simulink library "Yaw_Motor_Lib"  (R2025a)
settings: Solver=ode45  StartTime=0.0  StopTime=10.0  RelTol=1e-3  EnableMultiTasking=on
undefined symbols (not defined in the file): WT_Params
libraries: fl_lib x6, nesl_utility x5, ee_lib x1, sdl_lib x1, Yaw_Gearbox_Lib x1
Description:
  | Copyright 2009-2025 The MathWorks, Inc. MathWorks, Inc.
settings Model: Creator=smiller  LastModifiedBy=smiller
settings SolverCC: AlgebraicLoopSolver=TrustRegion
settings DataIOCC: LimitDataPoints=on  SaveFormat=Array  SignalLoggingSaveFormat=ModelDataLogs  ReturnWorkspaceOutputs=off
settings OptimizationCC: ReuseModelBlockBuffer=off  ExpressionDepthLimit=2147483647.0  LifeSpan=inf
settings DebuggingCC: UnderspecifiedInitializationDetection=Classic  MergeDetectMultiDrivingBlocksExec=none  SolverPrmCheckMsg=warning  FcnCallInpInsideContextMsg=warning  UnconnectedInputMsg=warning  UnconnectedOutputMsg=warning  UnconnectedLineMsg=warning  AllowSymbolicDim=off  StateNameClashWarn=warning  PregeneratedLibrarySubsystemCodeDiagnostic=none  SFUnexpectedBacktrackingDiag=warning  SFNoUnconditionalDefaultTransitionDiag=warning  SFExecutionAtInitializationDiag=none  ArithmeticOperatorsInVariantConditions=warning
settings HardwareCC: ProdBitPerPointer=32.0  ProdBitPerSizeT=32.0  ProdBitPerPtrDiffT=32.0  ProdLargestAtomicFloat=None  ProdIntDivRoundTo=Undefined  ProdEndianess=Unspecified  ProdWordSize=32.0  ProdHWDeviceType=32-bit Generic
settings ModelReferenceCC: EnableRefExpFcnMdlSchedulingChecks=on  PropagateSignalLabelsOutOfModel=off
settings SFSimCC: SimUseLocalCustomCode=off  CustomCodeUndefinedFunction=UseInterfaceOnly
settings RTWCC: RTWUseLocalCustomCode=off  GPUComputeCapability=3.5  DLArmComputeVersion=19.05
settings CodeAppCC: StateflowObjectComments=on
settings GRTTargetCC: TargetLangStandard=C89/C90 (ANSI)  CombineOutputUpdateFcns=off  GRTInterface=on
settings ConfigComp: CovMetricSettings=dw  CovSaveCumulativeToWorkspaceVar=on  CovSaveSingleToWorkspaceVar=on  CovExternalEMLEnable=off  CovSFcnEnable=off

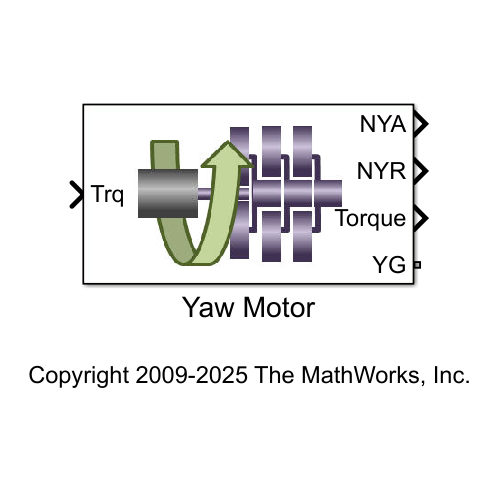
[thumbnail: Simulink's stored preview of the top-level diagram]
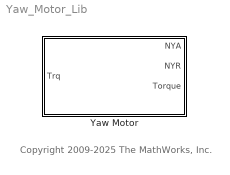
== system Yaw_Motor_Lib ==
  note: Copyright 2009-2025 The MathWorks, Inc.
  Yaw Motor : Subsystem
      mask Display: image('Yaw_Servomotor_Horizontal_IMAGE.jpg');

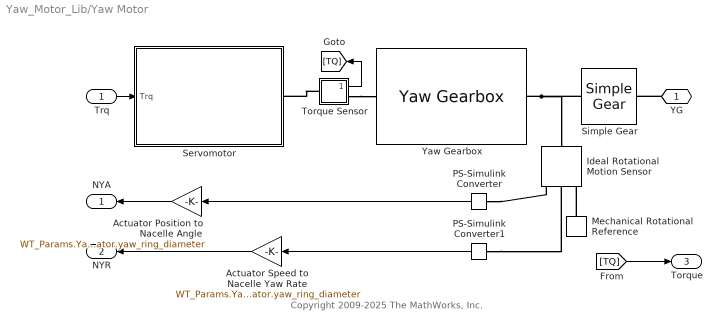
== system Yaw_Motor_Lib/Yaw Motor ==
  note: Copyright 2009-2025 The MathWorks, Inc.
  Trq : Inport
  Actuator Position to Nacelle Angle : Gain  Gain=WT_Params.Yaw_Actuator.yaw_gear_diameter/WT_Params.Yaw_Actuator.yaw_ring_diameter
  Actuator Speed to Nacelle Yaw Rate : Gain  Gain=WT_Params.Yaw_Actuator.yaw_gear_diameter/WT_Params.Yaw_Actuator.yaw_ring_diameter
  Ideal Rotational Motion Sensor : fl_lib/Mechanical/Mechanical Sensors/Ideal Rotational Motion Sensor  reference=foundation.enum.MeasurementReference.difference  acceleration_port=false  velocity_port=true  position_port=true  wrap_angle=simscape.enum.onoff.off  offset=0 rad
  Mechanical Rotational Reference : fl_lib/Mechanical/Rotational Elements/Mechanical Rotational Reference
  PS-Simulink Converter : nesl_utility/PS-Simulink Converter  PhysicalDomain=network_engine_domain  SubClassName=ps_output  LeftPortType=input  RightPortType=output  PseudoPeriodic=off  Frequencies=[]  VectorFormat=1-D array  Unit=deg  AffineConversion=off
  PS-Simulink Converter1 : nesl_utility/PS-Simulink Converter  PhysicalDomain=network_engine_domain  SubClassName=ps_output  LeftPortType=input  RightPortType=output  PseudoPeriodic=off  Frequencies=[]  VectorFormat=1-D array  Unit=deg/s  AffineConversion=off
  Servomotor : Subsystem
      mask Display: image(imread('Yaw_Servomotor_IMAGE.jpg'));
  Simple Gear : sdl_lib/Gears/Simple Gear  ratio=1/(WT_Params.Yaw_Actuator.yaw_gear_diameter/WT_Params.Yaw_Actuator.yaw_ring_diameter)  rotation_direction=3-2*(2)  friction_model=1  T_noload=0.1 N*m  T_nom=5 N*m  efficiency_nom=0.8  efficiency=0.8  temperature_TLU=[ 280 300 320 ] K  load_TLU=[ 1 5 10 ] N*m  efficiency_TLU=[ 0.95 0.9 0.85 ]  efficiency_TLU2=[ 0.85 0.8 0.75; 0.95 0.9 0.85; 0.85 0.8 0.7 ]  w_thr=0.01 rad/s  pwr_thr=0.001 W  enable_backlash=false  hardstop_model=simscape.enum.hardstop.smooth  backlash_distance=1e-3 mm  r_base=0.1 m  transition=1e-4 mm  backlash_stiffness=1e7 N/m  backlash_damping=1e6 N*s/m  coeff_rest=0  v_tol=0.001 m/s  f_tol=0 N  mu_visc=[ 0 0 ] N*m/(rad/s)  thermal_mass=50 J/K  temperature_specify=off  temperature_priority=High  temperature=300 K  temperature_nominal_specify=off  temperature_nominal_value=1  temperature_nominal_unit=K  x_backlash_specify=off  x_backlash_priority=None  x_backlash=0 mm  x_backlash_nominal_specify=off  x_backlash_nominal_value=1  x_backlash_nominal_unit=mm  f_hardstop_specify=off  f_hardstop_priority=None  f_hardstop=0 N  f_hardstop_nominal_specify=off  f_hardstop_nominal_value=1  f_hardstop_nominal_unit=N  v_backlash_specify=off  v_backlash_priority=None  v_backlash=0 m/s  v_backlash_nominal_specify=off  v_backlash_nominal_value=1  v_backlash_nominal_unit=m/s
  Torque Sensor : Subsystem
      mask Display: disp('S')
  Yaw Gearbox : Yaw_Gearbox_Lib/Yaw Gearbox  SystemSampleTime=-1  VariantActivationTime=update diagram  EmptyChoice=off  PassThrough=off  PassThroughVariantControl=(default)  EmptyChoiceVariantControl=(default)  AllowFlexibleInterface=on  Latency=0  AutoFrameSizeCalculation=off
  YG : PMIOPort  Side=Right
  NYA : Outport  VectorParamsAs1DForOutWhenUnconnected=off
  NYR : Outport  Port=2  VectorParamsAs1DForOutWhenUnconnected=off
  Torque : Outport  Port=3  VectorParamsAs1DForOutWhenUnconnected=off
  wires:
  PS-Simulink Converter1/1 -> Actuator Speed to Nacelle Yaw Rate/1
  PS-Simulink Converter/1 -> Actuator Position to Nacelle Angle/1
  [TQ] -> Torque/1
  Torque Sensor/1(Trq) -> [TQ]
  Actuator Speed to Nacelle Yaw Rate/1 -> NYR/1
  Actuator Position to Nacelle Angle/1 -> NYA/1
  Trq/1 -> Servomotor/1(Trq)
  connections:
  YG/RConn1 -- Simple Gear/RConn1
  PS-Simulink Converter/LConn1 -- Ideal Rotational Motion Sensor/RConn3
  Mechanical Rotational Reference/LConn1 -- Ideal Rotational Motion Sensor/RConn1
  PS-Simulink Converter1/LConn1 -- Ideal Rotational Motion Sensor/RConn2
  Yaw Gearbox/RConn1 -- Ideal Rotational Motion Sensor/LConn1 -- Simple Gear/LConn1
  Torque Sensor/RConn1 -- Yaw Gearbox/LConn1
  Torque Sensor/LConn1 -- Servomotor/RConn1

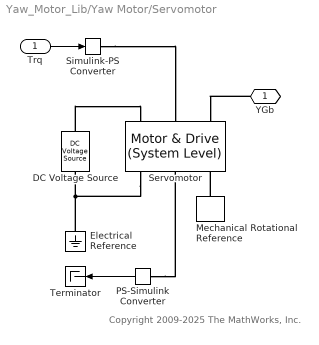
== system Yaw_Motor_Lib/Yaw Motor/Servomotor ==
  note: Copyright 2009-2025 The MathWorks, Inc.
  Trq : Inport
  DC Voltage Source : fl_lib/Electrical/Electrical Sources/DC Voltage Source  v0=WT_Params.Yaw_Actuator.Motor.voltage V
  Electrical Reference : fl_lib/Electrical/Electrical Elements/Electrical Reference
  Mechanical Rotational Reference : fl_lib/Mechanical/Rotational Elements/Mechanical Rotational Reference
  PS-Simulink Converter : nesl_utility/PS-Simulink Converter  PhysicalDomain=network_engine_domain  SubClassName=ps_output  LeftPortType=input  RightPortType=output  PseudoPeriodic=off  Frequencies=[]  VectorFormat=1-D array  Unit=deg/s  AffineConversion=off
  Servomotor : ee_lib/Electromechanical/Motor & Drive (System Level)  torque_speed_param=1  overtorque_param=ee.enum.electromech.overtorque.no  T_t=WT_Params.Yaw_Actuator.Motor.max_torque_vector N*m  T_t_intermittent=[.36, .32, .28, 0] N*m  T_t_2D=[.09, .09, .09; .08, .08, .08; .07, .07, .07; 0, 0, 0] N*m  T_t_intermittent_2D=[.36, .36, .36; .32, .32, .32; .28, .28, .28; 0, 0, 0] N*m  w_t=WT_Params.Yaw_Actuator.Motor.max_speed_vector rpm  vdc_t=[6, 12, 24] V  torque_max=0.1 N*m  power_max=30 W  torque_max_intermittent=0.4 N*m  power_max_intermittent=120 W  time_overtorque=30 s  time_recover=60 s  Tc=WT_Params.Yaw_Actuator.Motor.control_time_constant s  EnableSwitch=simscape.enum.onoff.off  losses_param=1  eff=100  w_eff=3.75e+03 rpm  T_eff=0.08 N*m  Piron=0 W  Pbase=0 W  w_eff_vec=[-8000 -4000 0 4000 8000] rpm  T_eff_vec=[0 0.03 0.06 0.09] N*m  v_eff_vec=[100, 250, 400] V  losses_mat=[1.49 1.67 2.21 3.10; 0.42 0.69 1.14 2.03; 0.06 0.24 0.78 1.68; 0.42 0.69 1.14 2.03; 1.49 1.67 2.21 3.10] W  efficiency_mat=[95 95 95 95; 95 95 95 95; 95 95 95 95; 95 95 95 95; 95 95 95 95]  losses_mat_3D=ones(5, 4, 3) W  efficiency_mat_3D=95 * ones(5, 4, 3)  Res=WT_Params.Yaw_Actuator.Motor.resistance Ohm  J=0 kg*m^2  lam=WT_Params.Yaw_Actuator.Motor.damping N*m/(rad/s)  speed0=0 rpm  faulted_specify=off  faulted_priority=None  faulted=0  faulted_nominal_specify=off  faulted_nominal_value=1  faulted_nominal_unit=1  isSwitchedOff_specify=off  isSwitchedOff_priority=None  isSwitchedOff=0  isSwitchedOff_nominal_specify=off  isSwitchedOff_nominal_value=1  isSwitchedOff_nominal_unit=1  torqueLimitContinuous_specify=off  torqueLimitContinuous_priority=None  torqueLimitContinuous=0 N*m  torqueLimitContinuous_nominal_specify=off  torqueLimitContinuous_nominal_value=1  torqueLimitContinuous_nominal_unit=N*m  alpha=3.93e-3 1/K  Tmeas=25 degC  Tmeas2=125 degC  losses_mat_T2=[1.49, 1.74, 2.49, 3.74; .42, .67, 1.42, 2.67; .06, .31, 1.06, 2.31; .42, .67, 1.42, 2.67; 1.49, 1.74, 2.49, 3.74] W  efficiency_mat_T2=[95, 95, 95, 95; 95, 95, 95, 95; 95, 95, 95, 95; 95, 95, 95, 95; 95, 95, 95, 95]  losses_mat_3D_T2=ones(5, 4, 3) W  efficiency_mat_3D_T2=95 * ones(5, 4, 3)  thermal_mass=100 J/K  initial_temperature=25 degC
  Simulink-PS Converter : nesl_utility/Simulink-PS Converter  PhysicalDomain=network_engine_domain  SubClassName=ps_input  LeftPortType=input  RightPortType=output  PseudoPeriodic=off  Frequencies=[]  NoiseDistribution=none  NoiseParameters=[]  Unit=1  AffineConversion=off  FilteringAndDerivatives=filter  SimscapeFilterOrder=1  InputFilterTimeConstant=0.005  UdotUserProvided=1
  Terminator : Terminator
  YGb : PMIOPort  Side=Right
  wires:
  Trq/1 -> Simulink-PS Converter/1
  PS-Simulink Converter/1 -> Terminator/1
  connections:
  YGb/RConn1 -- Servomotor/LConn3
  Simulink-PS Converter/RConn1 -- Servomotor/LConn2
  PS-Simulink Converter/LConn1 -- Servomotor/RConn2
  Mechanical Rotational Reference/LConn1 -- Servomotor/RConn3
  Electrical Reference/LConn1 -- DC Voltage Source/RConn1 -- Servomotor/RConn1
  DC Voltage Source/LConn1 -- Servomotor/LConn1

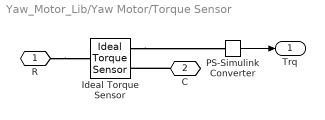
== system Yaw_Motor_Lib/Yaw Motor/Torque Sensor ==
  Ideal Torque Sensor : fl_lib/Mechanical/Mechanical Sensors/Ideal Torque Sensor
  PS-Simulink Converter : nesl_utility/PS-Simulink Converter  PhysicalDomain=network_engine_domain  SubClassName=ps_output  LeftPortType=input  RightPortType=output  PseudoPeriodic=off  Frequencies=[]  VectorFormat=1-D array  Unit=1  AffineConversion=off
  R : PMIOPort  Side=Left
  C : PMIOPort  Port=2  Side=Right
  Trq : Outport  VectorParamsAs1DForOutWhenUnconnected=off
  wires:
  PS-Simulink Converter/1 -> Trq/1
  connections:
  Ideal Torque Sensor/RConn2 -- PS-Simulink Converter/LConn1
  C/RConn1 -- Ideal Torque Sensor/RConn1
  R/RConn1 -- Ideal Torque Sensor/LConn1
